simulink model "Practica_6_simu"  (R2026a)
settings: Solver=FixedStepAuto  StopTime=0.01  FixedStep=1e-7

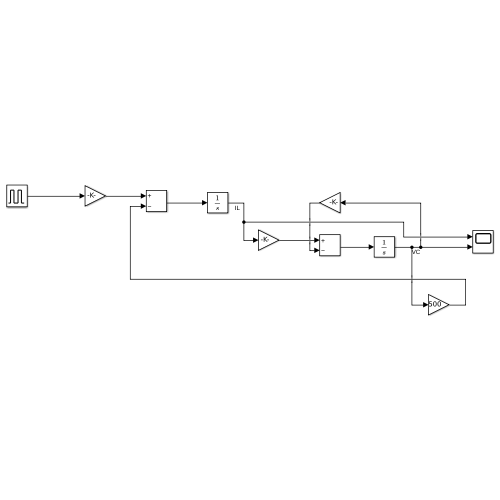
[thumbnail: Simulink's stored preview of the top-level diagram]
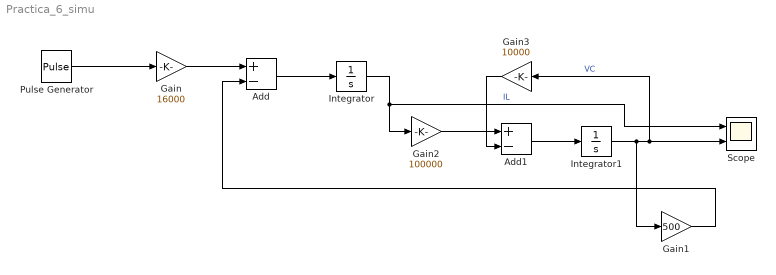
== system Practica_6_simu ==
  Add : Sum  Inputs=+-
  Add1 : Sum  Inputs=+-
  Gain : Gain  Gain=16000
  Gain1 : Gain  Gain=500
  Gain2 : Gain  Gain=100000
  Gain3 : Gain  Gain=10000
  Integrator : Integrator
  Integrator1 : Integrator
  Pulse Generator : DiscretePulseGenerator  PulseType=Time based  Period=1e-5  PulseWidth=40
  Scope : Scope  NumInputPorts=2
      settings: ActiveDisplayYMinimum=-1.6694297183254598  ActiveDisplayYMaximum=15.024867464929143
  wires:
  Pulse Generator/1 -> Gain/1
  Gain/1 -> Add/1
  Add/1 -> Integrator/1
  Gain2/1 -> Add1/1
  Add1/1 -> Integrator1/1
  Integrator/1 -> Scope/1, Gain2/1  "IL"
  Integrator1/1 -> Scope/2, Gain3/1, Gain1/1  "VC"
  Gain1/1 -> Add/2
  Gain3/1 -> Add1/2
